simulink model "AirplaneSimModel_LindiPlane"  (R2023b)
settings: Solver=ode1  StartTime=0.0  StopTime=60  FixedStep=1/400  RelTol=1e-3
undefined symbols (not defined in the file): aileron_left, aileron_right, airplane, alt_ground, atmosphere, elevator, envir, g, htp_trim, rudder, throttle, waypoints, wind
libraries: unit_conversions_lib x6, flightgear_visualization_lib x2, joystick_lib x1, conventional_airplane_single_engine_lib x1, atmosphere_lib x1, lindiPlane_lib x1, sensors_lib x1, simulink x1
settings Model: Creator=Fgücker  LastModifiedBy=yannic
settings SolverCC: AlgebraicLoopSolver=TrustRegion
settings DataIOCC: ReturnWorkspaceOutputs=off  LoggingToFile=on
settings DebuggingCC: UnconnectedInputMsg=warning  UnconnectedOutputMsg=warning  UnconnectedLineMsg=warning  ArithmeticOperatorsInVariantConditions=warning
settings ModelReferenceCC: EnableRefExpFcnMdlSchedulingChecks=on
settings SFSimCC: CustomCodeUndefinedFunction=UseInterfaceOnly

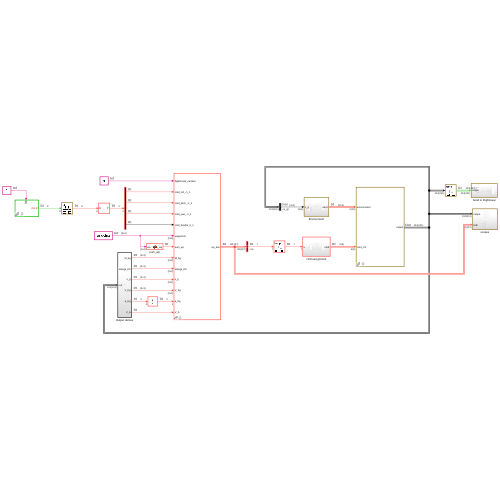
[thumbnail: Simulink's stored preview of the top-level diagram]
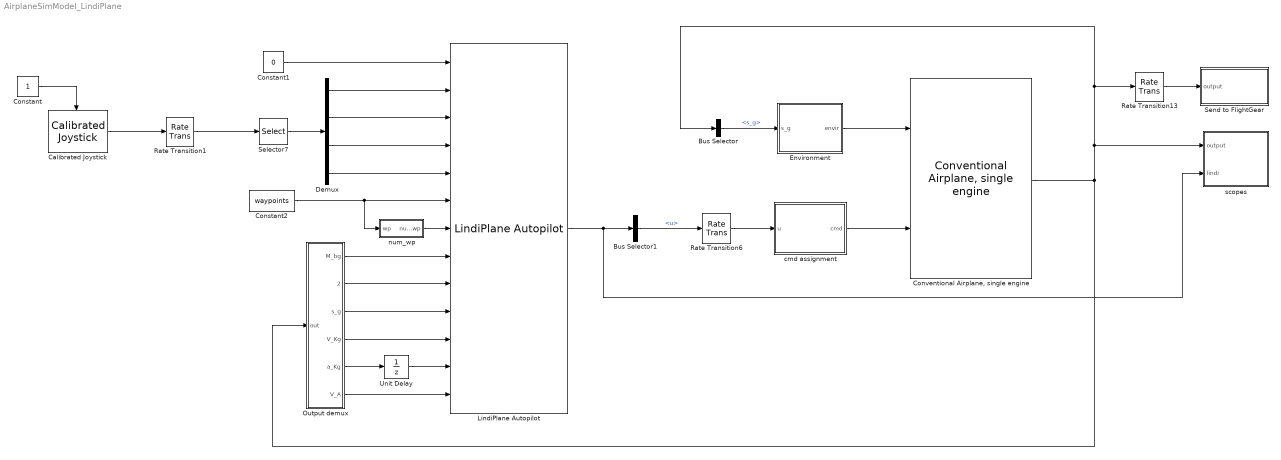
== system AirplaneSimModel_LindiPlane ==
  Bus Selector : BusSelector  OutputSignals=rigidBodyBus.s_g
  Bus Selector1 : BusSelector  OutputSignals=inner_loop_indi.u
  Calibrated Joystick : joystick_lib/Calibrated Joystick  jystck=jystck  joyid=1
      settings: SourceProductName=LADAC
  Constant : Constant
  Constant1 : Constant  Value=0
  Constant2 : Constant  Value=waypoints
  "Conventional Airplane, single engine" : conventional_airplane_single_engine_lib/Conventional Airplane, single engine  airplane=airplane
      settings: SourceProductName=LADAC
  Demux : Demux
  Environment : Subsystem
  LindiPlane Autopilot : lindiPlane_lib/LindiPlane Autopilot  ap=lindi  ap_notune=lindi_notune  is_enable_checked=off  states_when_enabling=reset  is_cmd_wrbm_n=off
  Output demux : Subsystem
  Rate Transition1 : RateTransition
  Rate Transition13 : RateTransition  OutPortSampleTime=1/50
  Rate Transition6 : RateTransition
  Selector7 : Selector  InputPortWidth=8  IndexOptions=Index vector (dialog)  Indices=[1:4]  OutputSizes=1
  Send to FlightGear : Subsystem
  Unit Delay : UnitDelay  SampleTime=-1  HasFrameUpgradeWarning=on
  cmd assignment : Subsystem
  num_wp : MATLAB Function  TreatAsAtomicUnit=on
  scopes : Subsystem
  wires:
  Environment/1(envir) -> "Conventional Airplane, single engine"/1
  Bus Selector/1 -> Environment/1(s_g)  "<s_g>"
  cmd assignment/1(cmd) -> "Conventional Airplane, single engine"/2
  Rate Transition6/1 -> cmd assignment/1(u)
  Rate Transition13/1 -> Send to FlightGear/1(output)
  Constant/1 -> Calibrated Joystick/Enable
  Calibrated Joystick/1 -> Rate Transition1/1
  Selector7/1 -> Demux/1
  Rate Transition1/1 -> Selector7/1
  Bus Selector1/1 -> Rate Transition6/1  "<u>"
  Constant1/1 -> LindiPlane Autopilot/1
  Demux/2 -> LindiPlane Autopilot/3
  Demux/3 -> LindiPlane Autopilot/4
  Constant2/1 -> LindiPlane Autopilot/6, num_wp/1(wp)
  num_wp/1(num_wp) -> LindiPlane Autopilot/7
  Demux/4 -> LindiPlane Autopilot/5
  "Conventional Airplane, single engine"/1 -> Output demux/1(out), Bus Selector/1, Rate Transition13/1, scopes/1(output)
  Output demux/1(M_bg) -> LindiPlane Autopilot/8
  Output demux/2(omega_Kb) -> LindiPlane Autopilot/9
  Output demux/3(s_g) -> LindiPlane Autopilot/10
  Output demux/4(V_Kg) -> LindiPlane Autopilot/11
  Output demux/6(V_A) -> LindiPlane Autopilot/13
  LindiPlane Autopilot/1 -> scopes/2(lindi), Bus Selector1/1
  Demux/1 -> LindiPlane Autopilot/2
  Output demux/5(a_Kg) -> Unit Delay/1
  Unit Delay/1 -> LindiPlane Autopilot/12

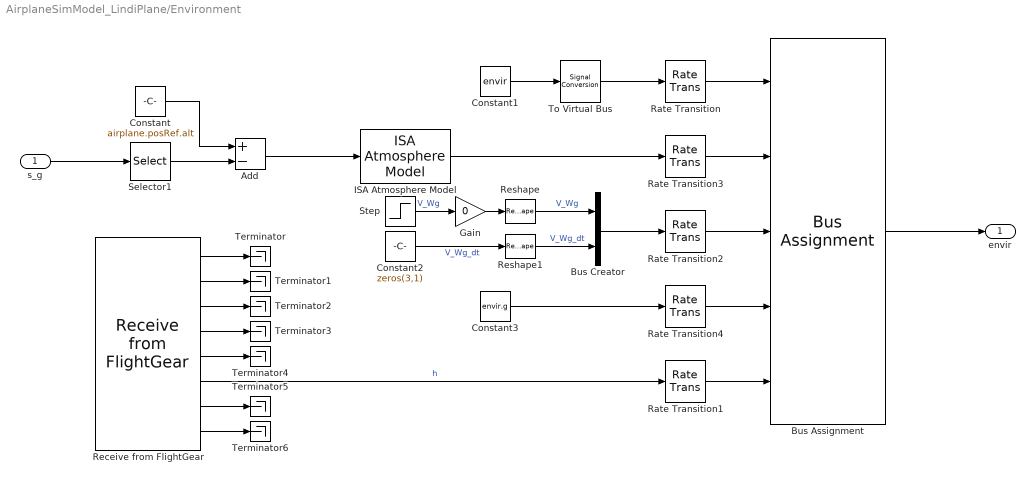
== system AirplaneSimModel_LindiPlane/Environment ==
  s_g : Inport
  Add : Sum  Inputs=+-
  Bus Assignment : BusAssignment  AssignedSignals=atmosphere,wind,g,alt_ground
  Bus Creator : BusCreator  Inputs=2
  Constant : Constant  Value=airplane.posRef.alt
  Constant1 : Constant  Value=envir  OutDataTypeStr=Bus: envirBus
  Constant2 : Constant  Value=zeros(3,1)
  Constant3 : Constant  Value=envir.g
  Gain : Gain  Gain=0
  ISA Atmosphere Model : atmosphere_lib/ISA Atmosphere Model
      settings: SourceProductName=LADAC
  Rate Transition{,1..4} (5 alike) : RateTransition
  Receive from FlightGear : flightgear_visualization_lib/Receive from FlightGear  ip_address='127.0.0.1'  ip_port=5503  sample_time=1/40  blocking_time=0  is_aerocntrl=off  is_engine=off  is_fuel=off  is_land=off  is_avionics=off  is_envir=on
      settings: SourceProductName=LADAC
  Reshape : Reshape  OutputDimensionality=Column vector (2-D)
  Reshape1 : Reshape  OutputDimensionality=Column vector (2-D)
  Selector1 : Selector  InputPortWidth=3  IndexOptions=Index vector (dialog)  Indices=3  OutputSizes=1
  Step : Step  Time=3  After=[0;9;0]  SampleTime=0
  Terminator{,1..6} (7 alike) : Terminator
  To Virtual Bus : SignalConversion  ConversionOutput=Virtual bus  OverrideOpt=off
  envir : Outport  VectorParamsAs1DForOutWhenUnconnected=off
  wires:
  Rate Transition2/1 -> Bus Assignment/3
  Rate Transition3/1 -> Bus Assignment/2
  Bus Assignment/1 -> envir/1
  Rate Transition/1 -> Bus Assignment/1
  ISA Atmosphere Model/1 -> Rate Transition3/1
  Step/1 -> Gain/1  "V_Wg"
  Rate Transition1/1 -> Bus Assignment/5
  Constant1/1 -> To Virtual Bus/1
  s_g/1 -> Selector1/1
  Bus Creator/1 -> Rate Transition2/1
  Constant2/1 -> Reshape1/1  "V_Wg_dt"
  Rate Transition4/1 -> Bus Assignment/4
  Constant3/1 -> Rate Transition4/1
  Gain/1 -> Reshape/1
  Constant/1 -> Add/1
  Add/1 -> ISA Atmosphere Model/1
  Selector1/1 -> Add/2
  To Virtual Bus/1 -> Rate Transition/1
  Reshape/1 -> Bus Creator/1  "V_Wg"
  Reshape1/1 -> Bus Creator/2  "V_Wg_dt"
  Receive from FlightGear/3 -> Terminator2/1
  Receive from FlightGear/1 -> Terminator/1
  Receive from FlightGear/6 -> Rate Transition1/1  "h"
  Receive from FlightGear/2 -> Terminator1/1
  Receive from FlightGear/5 -> Terminator4/1
  Receive from FlightGear/7 -> Terminator5/1
  Receive from FlightGear/4 -> Terminator3/1
  Receive from FlightGear/8 -> Terminator6/1

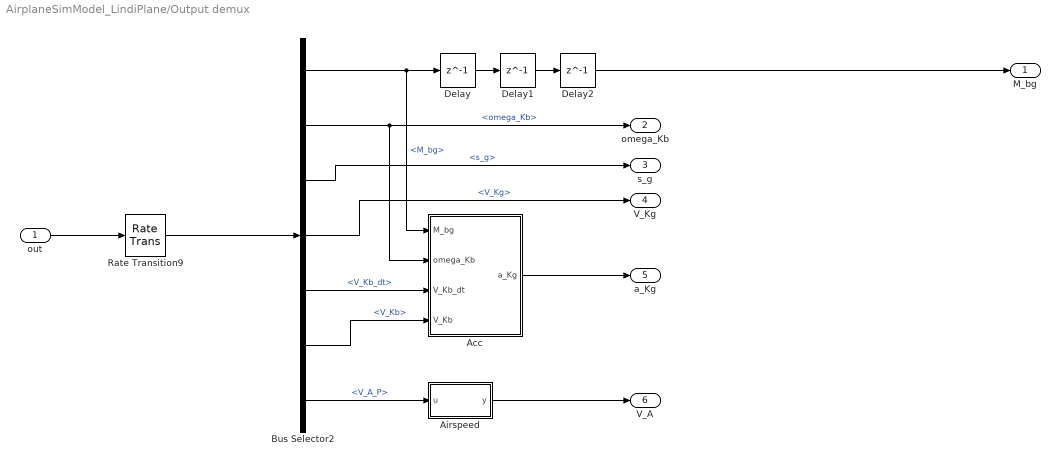
== system AirplaneSimModel_LindiPlane/Output demux ==
  out : Inport
  Acc : Subsystem
  Airspeed : MATLAB Function  TreatAsAtomicUnit=on
  Bus Selector2 : BusSelector  OutputSignals=rigidBodyBus.M_bg,rigidBodyBus.omega_Kb,rigidBodyBus.s_g,rigidBodyBus.V_Kg,rigidBodyBus.V_Kb_dt,rigidBodyBus.V_Kb,aeroBus.aeroMainWing.aeroAxes.V_A_P
  Delay : Delay  DelayLength=1  InitialCondition=eye(3)
  Delay1 : Delay  DelayLength=1  InitialCondition=eye(3)
  Delay2 : Delay  DelayLength=1  InitialCondition=eye(3)
  Rate Transition9 : RateTransition
  M_bg : Outport  VectorParamsAs1DForOutWhenUnconnected=off
  omega_Kb : Outport  Port=2  VectorParamsAs1DForOutWhenUnconnected=off
  s_g : Outport  Port=3  VectorParamsAs1DForOutWhenUnconnected=off
  V_Kg : Outport  Port=4  VectorParamsAs1DForOutWhenUnconnected=off
  a_Kg : Outport  Port=5  VectorParamsAs1DForOutWhenUnconnected=off
  V_A : Outport  Port=6  VectorParamsAs1DForOutWhenUnconnected=off
  wires:
  Bus Selector2/4 -> V_Kg/1  "<V_Kg>"
  Bus Selector2/6 -> Acc/4(V_Kb)  "<V_Kb>"
  Bus Selector2/1 -> Delay/1, Acc/1(M_bg)  "<M_bg>"
  Bus Selector2/5 -> Acc/3(V_Kb_dt)  "<V_Kb_dt>"
  Airspeed/1(y) -> V_A/1
  out/1 -> Rate Transition9/1
  Bus Selector2/3 -> s_g/1  "<s_g>"
  Bus Selector2/2 -> omega_Kb/1, Acc/2(omega_Kb)  "<omega_Kb>"
  Bus Selector2/7 -> Airspeed/1(u)  "<V_A_P>"
  Rate Transition9/1 -> Bus Selector2/1
  Acc/1(a_Kg) -> a_Kg/1
  Delay/1 -> Delay1/1
  Delay1/1 -> Delay2/1
  Delay2/1 -> M_bg/1

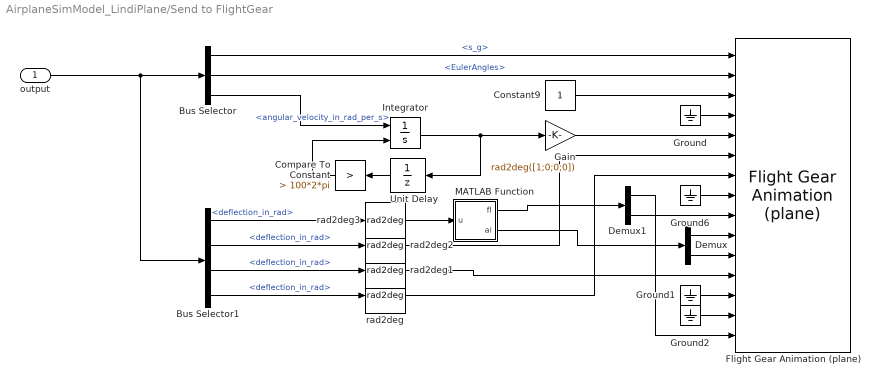
== system AirplaneSimModel_LindiPlane/Send to FlightGear ==
  output : Inport
  Bus Selector : BusSelector  OutputSignals=rigidBodyBus.s_g,rigidBodyBus.EulerAngles,actuatorBus.motorBus.angular_velocity_in_rad_per_s
  Bus Selector1 : BusSelector  OutputSignals=actuatorBus.aileronsBus.deflection_in_rad,actuatorBus.elevatorBus.deflection_in_rad,actuatorBus.rudderBus.deflection_in_rad,actuatorBus.htpTrimBus.deflection_in_rad
  Compare To Constant : simulink/Logic and Bit Operations/Compare To Constant  relop=>  const=100*2*pi  OutDataTypeStr=boolean
  Constant9 : Constant
  Demux : Demux  Outputs=2
  Demux1 : Demux  Outputs=2
  Flight Gear Animation (plane) : flightgear_visualization_lib/Flight Gear Animation (plane)  inital_lat=airplane.posRef.lat  inital_long=airplane.posRef.lon  inital_height=airplane.posRef.alt  remoteURL='127.0.0.1'  remotePort=5502
      settings: SourceProductName=LADAC
  Gain : Gain  Gain=rad2deg([1;0;0;0])
  Ground{,1..2,6} (4 alike) : Ground
  Integrator : Integrator  ExternalReset=rising
  MATLAB Function : MATLAB Function  TreatAsAtomicUnit=on
  Unit Delay : UnitDelay  SampleTime=-1  HasFrameUpgradeWarning=on
  rad2deg{,1..3} (4 alike) : unit_conversions_lib/rad2deg
      settings: SourceProductName=LADAC
  wires:
  Compare To Constant/1 -> Integrator/2
  Integrator/1 -> Unit Delay/1, Gain/1
  Bus Selector/1 -> Flight Gear Animation (plane)/1  "<s_g>"
  Bus Selector/2 -> Flight Gear Animation (plane)/2  "<EulerAngles>"
  Gain/1 -> Flight Gear Animation (plane)/5
  Constant9/1 -> Flight Gear Animation (plane)/3
  Unit Delay/1 -> Compare To Constant/1
  Ground/1 -> Flight Gear Animation (plane)/4
  Ground1/1 -> Flight Gear Animation (plane)/13
  Ground2/1 -> Flight Gear Animation (plane)/14
  Demux1/1 -> Flight Gear Animation (plane)/15
  output/1 -> Bus Selector1/1, Bus Selector/1
  Bus Selector/3 -> Integrator/1  "<angular_velocity_in_rad_per_s>"
  Bus Selector1/2 -> rad2deg2/1  "<deflection_in_rad>"
  Bus Selector1/4 -> rad2deg/1  "<deflection_in_rad>"
  Ground6/1 -> Flight Gear Animation (plane)/8
  Demux1/2 -> Flight Gear Animation (plane)/9
  Bus Selector1/3 -> rad2deg1/1  "<deflection_in_rad>"
  Bus Selector1/1 -> rad2deg3/1  "<deflection_in_rad>"
  Demux/1 -> Flight Gear Animation (plane)/10
  Demux/2 -> Flight Gear Animation (plane)/11
  rad2deg/1 -> Flight Gear Animation (plane)/7
  rad2deg1/1 -> Flight Gear Animation (plane)/12
  rad2deg2/1 -> Flight Gear Animation (plane)/6
  rad2deg3/1 -> MATLAB Function/1(u)
  MATLAB Function/2(ai) -> Demux/1
  MATLAB Function/1(fl) -> Demux1/1

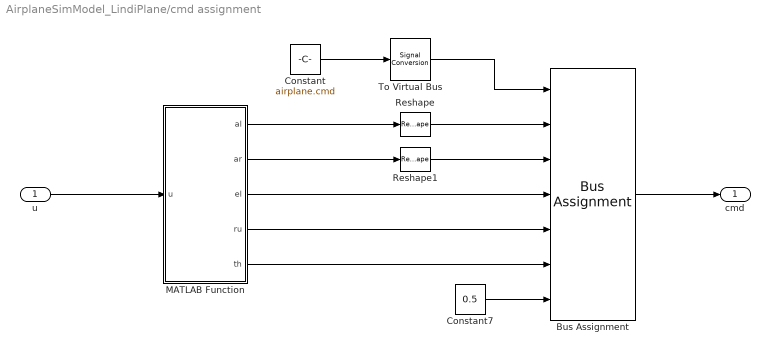
== system AirplaneSimModel_LindiPlane/cmd assignment ==
  u : Inport
  Bus Assignment : BusAssignment  AssignedSignals=aileron_left,aileron_right,elevator,rudder,throttle,htp_trim
  Constant : Constant  Value=airplane.cmd  OutDataTypeStr=Bus: cmdBus
  Constant7 : Constant  Value=0.5
  MATLAB Function : MATLAB Function  TreatAsAtomicUnit=on
  Reshape : Reshape  OutputDimensionality=Row vector (2-D)
  Reshape1 : Reshape  OutputDimensionality=Row vector (2-D)
  To Virtual Bus : SignalConversion  ConversionOutput=Virtual bus  OverrideOpt=off
  cmd : Outport  VectorParamsAs1DForOutWhenUnconnected=off
  wires:
  Constant/1 -> To Virtual Bus/1
  Bus Assignment/1 -> cmd/1
  Constant7/1 -> Bus Assignment/7
  u/1 -> MATLAB Function/1(u)
  MATLAB Function/3(el) -> Bus Assignment/4
  MATLAB Function/4(ru) -> Bus Assignment/5
  To Virtual Bus/1 -> Bus Assignment/1
  MATLAB Function/1(al) -> Reshape/1
  MATLAB Function/2(ar) -> Reshape1/1
  MATLAB Function/5(th) -> Bus Assignment/6
  Reshape/1 -> Bus Assignment/2
  Reshape1/1 -> Bus Assignment/3

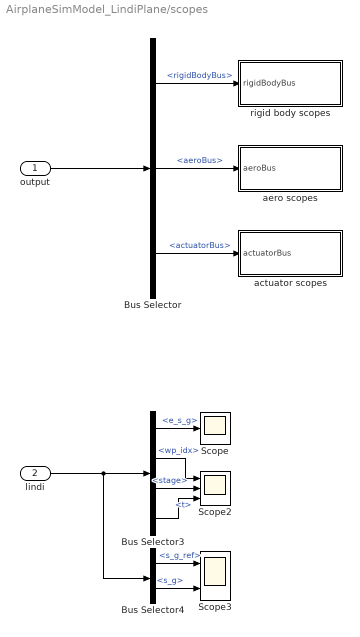
== system AirplaneSimModel_LindiPlane/scopes ==
  output : Inport
  lindi : Inport  Port=2
  Bus Selector : BusSelector  OutputSignals=rigidBodyBus,aeroBus,actuatorBus
  Bus Selector3 : BusSelector  OutputSignals=pos_control.error.e_s_g,wpnav.wp_idx,wpnav.stage,wpnav.t
  Bus Selector4 : BusSelector  OutputSignals=pos_control.reference.s_g_ref,pos_control.measure.s_g
  Scope : Scope
  Scope2 : Scope  NumInputPorts=3
  Scope3 : Scope  NumInputPorts=2
  actuator scopes : Subsystem
  aero scopes : Subsystem
  rigid body scopes : Subsystem
  wires:
  Bus Selector/1 -> rigid body scopes/1(rigidBodyBus)  "<rigidBodyBus>"
  Bus Selector/2 -> aero scopes/1(aeroBus)  "<aeroBus>"
  output/1 -> Bus Selector/1
  Bus Selector/3 -> actuator scopes/1(actuatorBus)  "<actuatorBus>"
  Bus Selector3/4 -> Scope2/3  "<t>"
  Bus Selector3/3 -> Scope2/2  "<stage>"
  Bus Selector3/2 -> Scope2/1  "<wp_idx>"
  Bus Selector4/1 -> Scope3/1  "<s_g_ref>"
  Bus Selector4/2 -> Scope3/2  "<s_g>"
  Bus Selector3/1 -> Scope/1  "<e_s_g>"
  lindi/1 -> Bus Selector4/1, Bus Selector3/1

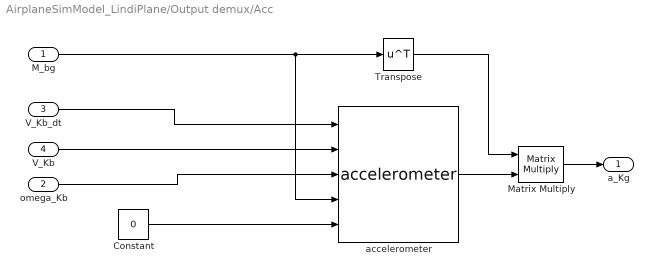
== system AirplaneSimModel_LindiPlane/Output demux/Acc ==
  M_bg : Inport
  omega_Kb : Inport  Port=2
  V_Kb_dt : Inport  Port=3
  V_Kb : Inport  Port=4
  Constant : Constant  Value=0  OutDataTypeStr=Inherit: Inherit via back propagation
  Matrix Multiply : Product  Multiplication=Matrix(*)
  Transpose : Math  Operator=transpose  SignedPower=on
  accelerometer : sensors_lib/accelerometer  SystemSampleTime=-1  VariantActivationTime=update diagram  AllowFlexibleInterface=on  Latency=0  AutoFrameSizeCalculation=off
      settings: SourceProductName=LADAC
  a_Kg : Outport  VectorParamsAs1DForOutWhenUnconnected=off
  wires:
  Transpose/1 -> Matrix Multiply/1
  V_Kb_dt/1 -> accelerometer/1
  omega_Kb/1 -> accelerometer/3
  accelerometer/1 -> Matrix Multiply/2
  Constant/1 -> accelerometer/5
  V_Kb/1 -> accelerometer/2
  M_bg/1 -> Transpose/1, accelerometer/4
  Matrix Multiply/1 -> a_Kg/1

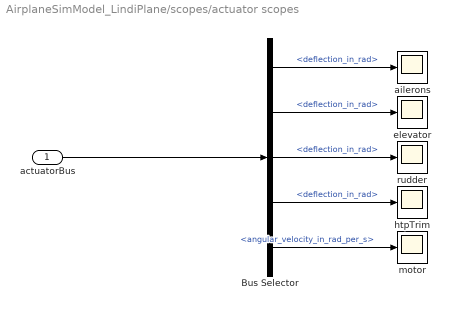
== system AirplaneSimModel_LindiPlane/scopes/actuator scopes ==
  actuatorBus : Inport
  Bus Selector : BusSelector  OutputSignals=aileronsBus.deflection_in_rad,elevatorBus.deflection_in_rad,rudderBus.deflection_in_rad,htpTrimBus.deflection_in_rad,motorBus.angular_velocity_in_rad_per_s
  ailerons : Scope
  elevator : Scope
  htpTrim : Scope
  motor : Scope
  rudder : Scope
  wires:
  actuatorBus/1 -> Bus Selector/1
  Bus Selector/1 -> ailerons/1  "<deflection_in_rad>"
  Bus Selector/2 -> elevator/1  "<deflection_in_rad>"
  Bus Selector/3 -> rudder/1  "<deflection_in_rad>"
  Bus Selector/4 -> htpTrim/1  "<deflection_in_rad>"
  Bus Selector/5 -> motor/1  "<angular_velocity_in_rad_per_s>"

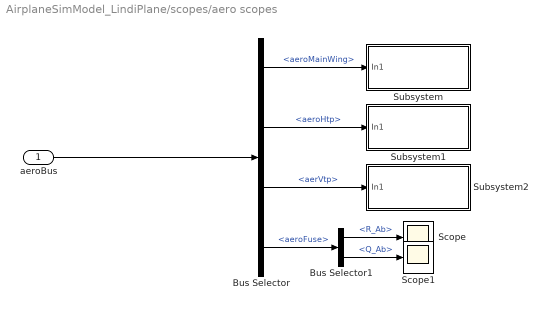
== system AirplaneSimModel_LindiPlane/scopes/aero scopes ==
  aeroBus : Inport
  Bus Selector : BusSelector  OutputSignals=aeroMainWing,aeroHtp,aerVtp,aeroFuse
  Bus Selector1 : BusSelector  OutputSignals=R_Ab,Q_Ab
  Scope : Scope
  Scope1 : Scope
  Subsystem : Subsystem
  Subsystem1 : Subsystem
  Subsystem2 : Subsystem
  wires:
  aeroBus/1 -> Bus Selector/1
  Bus Selector/1 -> Subsystem/1(In1)  "<aeroMainWing>"
  Bus Selector/2 -> Subsystem1/1(In1)  "<aeroHtp>"
  Bus Selector/3 -> Subsystem2/1(In1)  "<aerVtp>"
  Bus Selector/4 -> Bus Selector1/1  "<aeroFuse>"
  Bus Selector1/1 -> Scope/1  "<R_Ab>"
  Bus Selector1/2 -> Scope1/1  "<Q_Ab>"

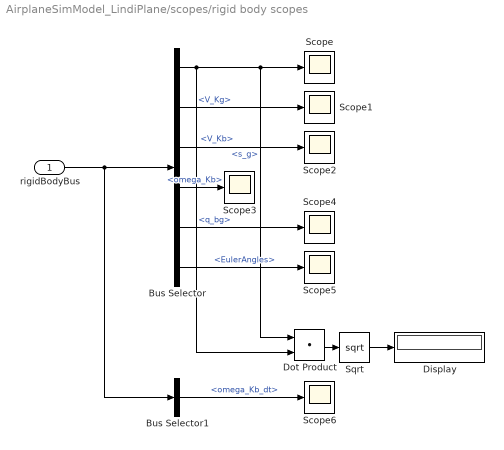
== system AirplaneSimModel_LindiPlane/scopes/rigid body scopes ==
  rigidBodyBus : Inport
  Bus Selector : BusSelector  OutputSignals=V_Kb,V_Kg,s_g,omega_Kb,q_bg,EulerAngles
  Bus Selector1 : BusSelector  OutputSignals=omega_Kb_dt
  Display : Display
  Dot Product : DotProduct  OutDataTypeStr=Inherit: Inherit via internal rule
  Scope{,1..6} (7 alike) : Scope
  Sqrt : Sqrt
  wires:
  rigidBodyBus/1 -> Bus Selector1/1, Bus Selector/1
  Bus Selector/1 -> Dot Product/1, Scope/1, Dot Product/2  "<V_Kb>"
  Bus Selector/2 -> Scope1/1  "<V_Kg>"
  Bus Selector/3 -> Scope2/1  "<s_g>"
  Bus Selector/4 -> Scope3/1  "<omega_Kb>"
  Bus Selector/5 -> Scope4/1  "<q_bg>"
  Bus Selector/6 -> Scope5/1  "<EulerAngles>"
  Dot Product/1 -> Sqrt/1
  Sqrt/1 -> Display/1
  Bus Selector1/1 -> Scope6/1  "<omega_Kb_dt>"

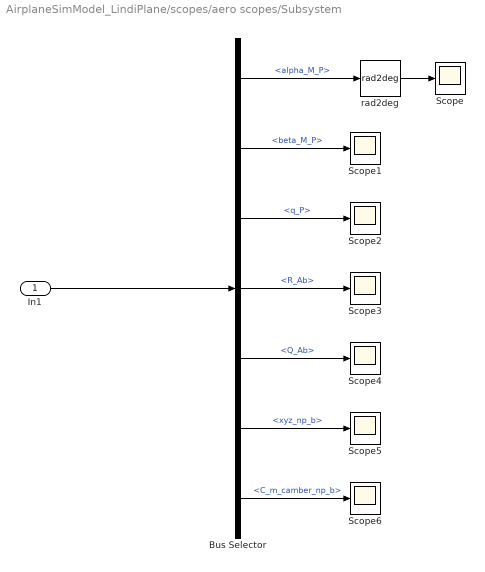
== system AirplaneSimModel_LindiPlane/scopes/aero scopes/Subsystem ==
  In1 : Inport
  Bus Selector : BusSelector  OutputSignals=aeroAxes.alpha_M_P,aeroAxes.beta_M_P,aeroAxes.q_P,dynamicsBody.R_Ab,dynamicsBody.Q_Ab,dynamicsBody.xyz_np_b,dynamicsBody.C_m_camber_np_b
  Scope{,1..6} (7 alike) : Scope
  rad2deg : unit_conversions_lib/rad2deg
      settings: SourceProductName=LADAC
  wires:
  Bus Selector/1 -> rad2deg/1  "<alpha_M_P>"
  Bus Selector/3 -> Scope2/1  "<q_P>"
  Bus Selector/2 -> Scope1/1  "<beta_M_P>"
  Bus Selector/4 -> Scope3/1  "<R_Ab>"
  Bus Selector/5 -> Scope4/1  "<Q_Ab>"
  Bus Selector/6 -> Scope5/1  "<xyz_np_b>"
  Bus Selector/7 -> Scope6/1  "<C_m_camber_np_b>"
  rad2deg/1 -> Scope/1
  In1/1 -> Bus Selector/1

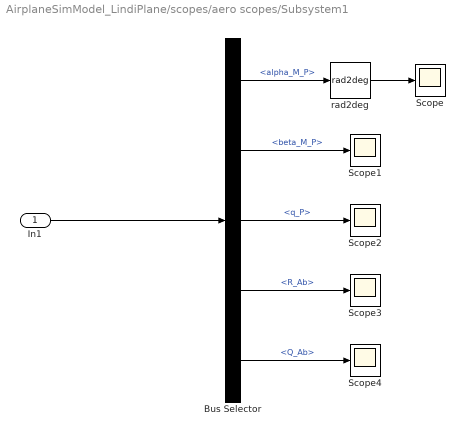
== system AirplaneSimModel_LindiPlane/scopes/aero scopes/Subsystem1 ==
  In1 : Inport
  Bus Selector : BusSelector  OutputSignals=aeroAxes.alpha_M_P,aeroAxes.beta_M_P,aeroAxes.q_P,dynamicsBody.R_Ab,dynamicsBody.Q_Ab
  Scope{,1..4} (5 alike) : Scope
  rad2deg : unit_conversions_lib/rad2deg
      settings: SourceProductName=LADAC
  wires:
  Bus Selector/5 -> Scope4/1  "<Q_Ab>"
  Bus Selector/4 -> Scope3/1  "<R_Ab>"
  Bus Selector/2 -> Scope1/1  "<beta_M_P>"
  Bus Selector/3 -> Scope2/1  "<q_P>"
  Bus Selector/1 -> rad2deg/1  "<alpha_M_P>"
  In1/1 -> Bus Selector/1
  rad2deg/1 -> Scope/1

== system AirplaneSimModel_LindiPlane/scopes/aero scopes/Subsystem2 ==
  In1 : Inport
  Bus Selector : BusSelector  OutputSignals=aeroAxes.alpha_M_P,aeroAxes.beta_M_P,aeroAxes.q_P,dynamicsBody.R_Ab,dynamicsBody.Q_Ab
  Scope{,1..4} (5 alike) : Scope
  wires:
  In1/1 -> Bus Selector/1
  Bus Selector/1 -> Scope/1  "<alpha_M_P>"
  Bus Selector/3 -> Scope2/1  "<q_P>"
  Bus Selector/2 -> Scope1/1  "<beta_M_P>"
  Bus Selector/4 -> Scope3/1  "<R_Ab>"
  Bus Selector/5 -> Scope4/1  "<Q_Ab>"

== matlab function AirplaneSimModel_LindiPlane/Output demux/Airspeed ==
  data: u input; y output
function y = fcn(u)
y = mean(u);
end

== matlab function AirplaneSimModel_LindiPlane/Send to FlightGear/MATLAB Function ==
  data: u input; fl output; ai output
function [fl,ai] = fcn(u)
ai = u([1,end]);
fl = [0,0];
if length(u)>=4
    fl(:) = u([end/2,end/2+1]);
end
end

== matlab function AirplaneSimModel_LindiPlane/cmd assignment/MATLAB Function ==
  data: u input; al output; ar output; el output; ru output; th output
function [al,ar,el,ru,th] = fcn(u)
ai = u(1:end-3) * 0.5 + 0.5;
al = ai(1:end/2);
ar = ai(end/2+1:end);
el = u(end-2) * 0.5 + 0.5;
ru = u(end-1) * 0.5 + 0.5;
th = u(end);
end

== matlab function AirplaneSimModel_LindiPlane/num_wp ==
  data: wp input; num_wp output
function num_wp = fcn(wp)
num_wp = size(wp,2);
end
